simulink model "FullSystem_Electrical_Testbench"  (R2025b)
settings: Solver=ode23t  StartTime=0.0  StopTime=inf  FixedStep=Ts  MaxStep=0.0001  RelTol=1e-3
values from neighbouring files (symbols this model uses):
  servoVelocityKi = servoWn.^2.*servoJeq    [init_servos.m]
  servoVelocityKp = 2*servoZeta.*servoWn.*servoJeq    [init_servos.m]
  Ts = 0.002    [init_trajectory.m]
libraries: simulink x2
settings Model: SimulationMode=accelerator  Creator=Compu  LastModifiedBy=Compu
settings SolverCC: ZeroCrossAlgorithm=Adaptive
settings DebuggingCC: UnconnectedInputMsg=warning  UnconnectedOutputMsg=warning  UnconnectedLineMsg=warning
settings ExplorerConfigSet: SimMechanicsOpenEditorOnUpdate=off

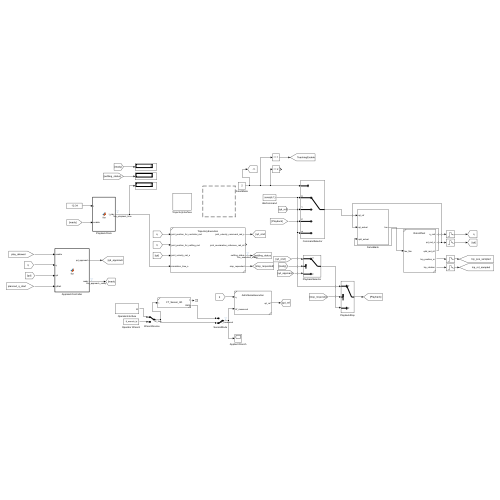
[thumbnail: Simulink's stored preview of the top-level diagram]
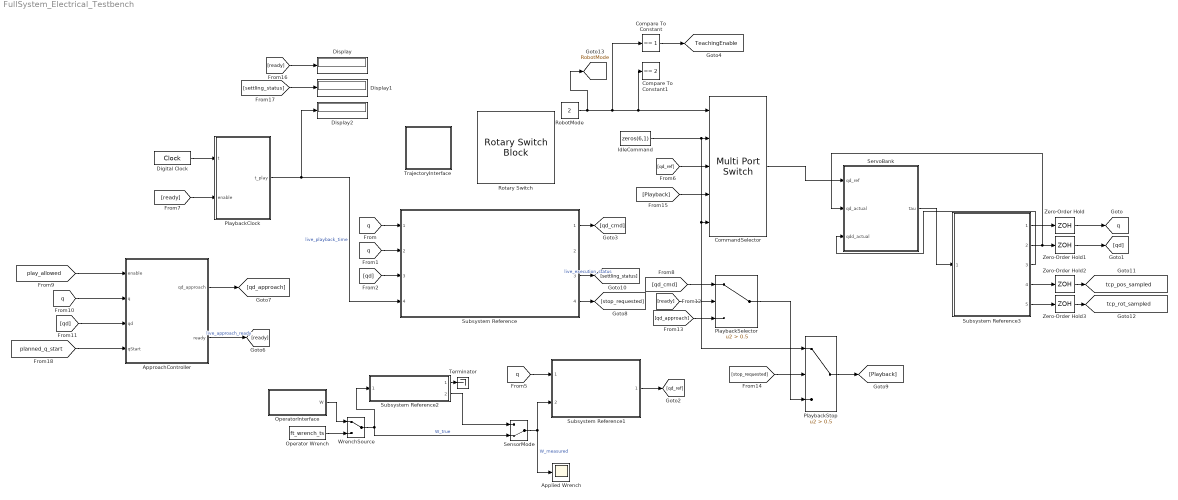
== system FullSystem_Electrical_Testbench ==
  Applied Wrench : Scope
      settings: DataLoggingVariableName=ScopeData3
  ApproachController : MATLAB Function  TreatAsAtomicUnit=on
  CommandSelector : MultiPortSwitch  DataPortOrder=Zero-based contiguous  DataPortForDefault=Additional data port  zeroidx=on  SaturateOnIntegerOverflow=off  InputSameDT=off
  Compare To Constant : simulink/Logic and Bit Operations/Compare To Constant  relop===  const=1  OutDataTypeStr=boolean
  Compare To Constant1 : simulink/Logic and Bit Operations/Compare To Constant  relop===  const=2  OutDataTypeStr=boolean
  Digital Clock : DigitalClock  SampleTime=Ts
  Display : Display
  Display1 : Display
  Display2 : Display
  IdleCommand : Constant  Value=zeros(6,1)  SampleTime=Ts
  Operator Wrench : FromWorkspace  VariableName=ft_wrench_ts  SampleTime=Ts  Interpolate=off  OutputAfterFinalValue=Holding final value
  OperatorInterface : Subsystem
  PlaybackClock : MATLAB Function  TreatAsAtomicUnit=on
  PlaybackSelector : Switch  Criteria=u2 > Threshold  Threshold=0.5  SaturateOnIntegerOverflow=off  InputSameDT=off
  PlaybackStop : Switch  Criteria=u2 > Threshold  Threshold=0.5  SaturateOnIntegerOverflow=off  InputSameDT=off
  RobotMode : Constant  Value=2  SampleTime=Ts
  Rotary Switch : RotarySwitchBlock
  SensorMode : ManualSwitch  CurrentSetting=0
  ServoBank : Subsystem
  Subsystem Reference : Subsystem  ReferencedSubsystem=TrajectoryExecution
  Subsystem Reference1 : Subsystem  ReferencedSubsystem=AdmittanceExecution
  Subsystem Reference2 : Subsystem  ReferencedSubsystem=FT_Sensor_6D
  Subsystem Reference3 : Subsystem  ReferencedSubsystem=RobotPlant
  Terminator : Terminator
  TrajectoryInterface : Subsystem
  WrenchSource : ManualSwitch
  Zero-Order Hold{,1..3} (4 alike) : ZeroOrderHold  SampleTime=Ts
  tag scope: RobotMode=global, TeachingEnable=global, q=global, tcp_pos_sampled=global, tcp_rot_sampled=global
  wires:
  Subsystem Reference2/2 -> SensorMode/1
  SensorMode/1 -> Subsystem Reference1/2, Applied Wrench/1  "W_measured"
  OperatorInterface/1(W) -> WrenchSource/1
  WrenchSource/1 -> SensorMode/2, Subsystem Reference2/1  "W_true"
  Subsystem Reference2/1 -> Terminator/1
  Operator Wrench/1 -> WrenchSource/2
  ServoBank/1(tau) -> Subsystem Reference3/1
  Subsystem Reference3/1 -> Zero-Order Hold/1
  Subsystem Reference3/2 -> ServoBank/2(qd_actual), Zero-Order Hold1/1
  Zero-Order Hold/1 -> [q]
  Zero-Order Hold1/1 -> [qd]
  [q] -> Subsystem Reference/1
  [q] -> Subsystem Reference/2
  [qd] -> Subsystem Reference/3
  [q] -> Subsystem Reference1/1
  RobotMode/1 -> [RobotMode], Compare To Constant/1, Compare To Constant1/1, CommandSelector/1
  Subsystem Reference1/1 -> [qd_ref]
  Subsystem Reference/1 -> [qd_cmd]
  [qd_ref] -> CommandSelector/3
  CommandSelector/1 -> ServoBank/1(qd_ref)
  Compare To Constant/1 -> [TeachingEnable]
  PlaybackClock/1(t_play) -> Display2/1, Subsystem Reference/4  "live_playback_time"
  Digital Clock/1 -> PlaybackClock/1(t)
  [q] -> ApproachController/2(q)
  [qd] -> ApproachController/3(qd)
  [play_allowed] -> ApproachController/1(enable)
  [planned_q_start] -> ApproachController/4(qStart)
  [qd_cmd] -> PlaybackSelector/1
  ApproachController/2(ready) -> [ready]  "live_approach_ready"
  ApproachController/1(qd_approach) -> [qd_approach]
  [ready] -> PlaybackClock/2(enable)
  [ready] -> PlaybackSelector/2
  [qd_approach] -> PlaybackSelector/3
  IdleCommand/1 -> CommandSelector/2, CommandSelector/5, PlaybackStop/1
  Subsystem Reference/4 -> [stop_requested]
  [stop_requested] -> PlaybackStop/2
  PlaybackSelector/1 -> PlaybackStop/3
  PlaybackStop/1 -> [Playback]
  [Playback] -> CommandSelector/4
  Subsystem Reference/3 -> [settling_status]  "live_execution_status"
  [ready] -> Display/1
  [settling_status] -> Display1/1
  Subsystem Reference3/4 -> Zero-Order Hold2/1
  Subsystem Reference3/5 -> Zero-Order Hold3/1
  Zero-Order Hold2/1 -> [tcp_pos_sampled]
  Zero-Order Hold3/1 -> [tcp_rot_sampled]
  Subsystem Reference3/3 -> ServoBank/3(qdd_actual)

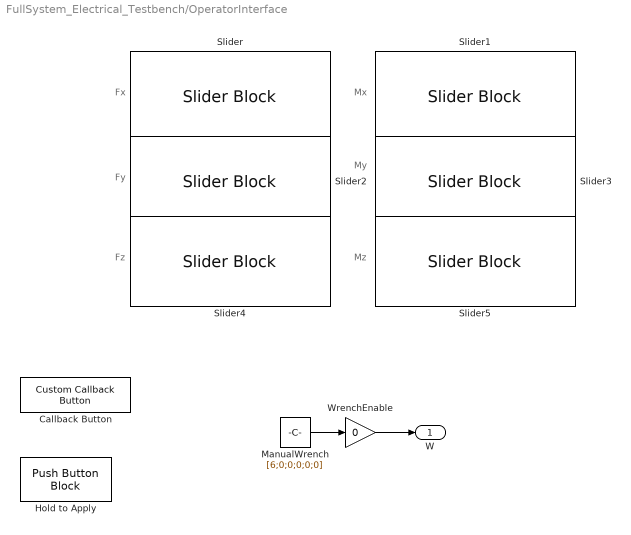
== system FullSystem_Electrical_Testbench/OperatorInterface ==
  note: Fx
  note: Fy
  note: Fz
  note: Mx
  note: My
  note: Mz
  Callback Button : CustomCallbackButton  Configuration="{\"components\":[{\"name\":\"BackgroundImageComponent\",\"settings\":{\"image\":{\"size\":[0,0],\"src\":\"default\",\"srcOrientation\":\"Right\"},\"position\":[0,0,1,1]}},{\"name\":\"ButtonStateComponent\",\"settings\":{\"buttonType\":\"momentary\",\"clickFcn\":\"set_param([get_param(gcb,'Parent') '\\/ManualWrench'], 'Value', '[0;0;0;0;0;0]');\",\"onValue\":1,\"position\":[0,0,1,1],\"pressDelay\":\"500\",\"pressFcn\":\"\",\"repeatInterval\":\"0\",\"states\":[{\"horizontalAlignment\":\"center\",\"image\":{\"position\":[0,0,1,1],\"size\":[1,1],\"src\":\"default\",\"srcOrientation\":\"Right\"},\"label\":{\"color\":[0.01176470588,0.01176470588,0.01176470588,1],\"icon\":{\"size\":[0,0],\"src\":\"default\",\"srcOrientation\":\"Right\"},\"iconOffset\":0,\"iconPlacement\":\"left\",\"opacity\":1,\"show\":true,\"text\":{\"content\":\"Reset All\",\"font\":\"Helvetica\"}},\"labelOffset\":[0,0],\"verticalAlignment\":\"middle\"},{\"horizontalAlignment\":\"center\",\"image\":{\"position\":[0,0,1,1],\"size\":[1,1],\"src\":\"default\",\"srcOrientation\":\"Right\"},\"label\":{\"color\":[0.01176470588,0.01176470588,0.01176470588,1],\"icon\":{\"size\":[0,0],\"src\":\"default\",\"srcOrientation\":\"Right\"},\"iconOffset\":0,\"iconPlacement\":\"left\",\"opacity\":1,\"show\":true,\"text\":{\"content\":\"Reset All\",\"font\":\"Helvetica\"}},\"labelOffset\":[0,0],\"verticalAlignment\":\"middle\"},{\"horizontalAlignment\":\"center\",\"image\":{\"position\":[0,0,1,1],\"size\":[1,1],\"src\":\"default\",\"srcOrientation\":\"Right\"},\"label\":{\"color\":[0.01176470588,0.01176470588,0.01176470588,1],\"icon\":{\"size\":[0,0],\"src\":\"default\",\"srcOrientation\":\"Right\"},\"iconOffset\":0,\"iconPlacement\":\"left\",\"opacity\":1,\"show\":true,\"text\":{\"content\":\"Reset All\",\"font\":\"Helvetica\"}},\"labelOffset\":[0,0],\"verticalAlignment\":\"middle\"},{\"horizontalAlignment\":\"center\",\"image\":{\"position\":[0,0,1,1],\"size\":[1,1],\"src\":\"default\",\"srcOrientation\":\"Right\"},\"label\":{\"color\":[0.01176470588,0.01176470588,0.01176470588,1],\"icon\":{\"size\":[0,0],\"src\":\"default\",\"srcOrientation\":\"Right\"},\"iconOffset\":0,\"iconPlacement\":\"left\",\"opacity\":1,\"show\":true,\"text\":{\"content\":\"Reset All\",\"font\":\"Helvetica\"}},\"labelOffset\":[0,0],\"verticalAlignment\":\"middle\"}]}},{\"name\":\"ForegroundImageComponent\",\"settings\":{\"image\":{\"size\":[0,0],\"src\":\"default\",\"srcOrientation\":\"Right\"},\"isForeground\":1,\"position\":[0,0,1,1]}}],\"derived\":{\"blockParameters\":{\"AutoActivate\":true,\"ButtonText\":\"Reset All\",\"ButtonType\":\"Momentary\",\"ClickFcn\":\"set_param([get_param(gcb,'Parent') '\\/ManualWrench'], 'Value', '[0;0;0;0;0;0]');\",\"OnValue\":1,\"PressDelay\":\"500\",\"PressFcn\":\"\",\"RepeatInterval\":\"0\",\"fixedAspectRatio\":\"off\"}},\"settings\":{\"BindingType\":\"standalone\",\"autoActivate\":true,\"backgroundColor\":[244,244,244,1],\"backgroundOffset\":0.2,\"backgroundOpacity\":1,\"fixedAspectRatio\":\"off\",\"foregroundColor\":[0.01176470588,0.01176470588,0.01176470588,1],\"migratedFromLegacy\":true,\"useBackgroundColor\":true,\"variant\":\"callback\",\"version\":\"R2025a\"},\"type\":\"Button\"}"  CustomBackgroundColor="{\"color\":[0.9568627451,0.9568627451,0.9568627451],\"show\":true}"
  Hold to Apply : PushButtonBlock  ButtonText=Hold to Apply  IconOnColor=[0.0, 0.39215686274509803, 0.0]  IconOffColor=[0.0, 1.0, 0.0]  OffValue=0.000000
  ManualWrench : Constant  Value=[6;0;0;0;0;0]  SampleTime=Ts
  Slider : SliderBlock  ScaleMin=-10  ScaleMax=10  TickInterval=5
  Slider1 : SliderBlock  ScaleMin=-1  ScaleMax=1  TickInterval=0.5
  Slider2 : SliderBlock  ScaleMin=-10  ScaleMax=10  TickInterval=5
  Slider3 : SliderBlock  ScaleMin=-1  ScaleMax=1  TickInterval=0.5
  Slider4 : SliderBlock  ScaleMin=-10  ScaleMax=10  TickInterval=5
  Slider5 : SliderBlock  ScaleMin=-1  ScaleMax=1  TickInterval=0.5
  WrenchEnable : Gain  Gain=0
  W : Outport
  wires:
  ManualWrench/1 -> WrenchEnable/1
  WrenchEnable/1 -> W/1

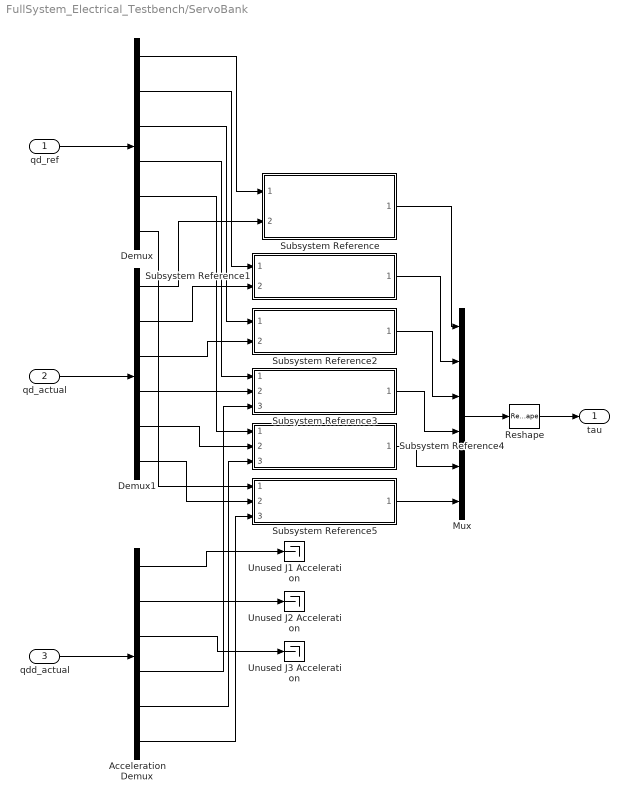
== system FullSystem_Electrical_Testbench/ServoBank ==
  qd_ref : Inport
  qd_actual : Inport  Port=2
  qdd_actual : Inport  Port=3
  Acceleration Demux : Demux  Outputs=6
  Demux : Demux  Outputs=6
  Demux1 : Demux  Outputs=6
  Mux : Mux  Inputs=6
  Reshape : Reshape  OutputDimensionality=Column vector (2-D)
  Subsystem Reference : Subsystem  ReferencedSubsystem=M8010_Actuator  VelKp=servoVelocityKp(1)  VelKi=servoVelocityKi(1)
  Subsystem Reference1 : Subsystem  ReferencedSubsystem=M8025_Actuator  VelKp=servoVelocityKp(2)  VelKi=servoVelocityKi(2)
  Subsystem Reference2 : Subsystem  ReferencedSubsystem=M8010_Actuator  VelKp=servoVelocityKp(3)  VelKi=servoVelocityKi(3)
  Subsystem Reference3 : Subsystem  ReferencedSubsystem=M6030G9_Actuator  VelKp=servoVelocityKp(4)  VelKi=servoVelocityKi(4)
  Subsystem Reference4 : Subsystem  ReferencedSubsystem=M6030G9_Actuator  VelKp=servoVelocityKp(5)  VelKi=servoVelocityKi(5)
  Subsystem Reference5 : Subsystem  ReferencedSubsystem=M6030G9_Actuator  VelKp=servoVelocityKp(6)  VelKi=servoVelocityKi(6)
  Unused J1 Acceleration : Terminator
  Unused J2 Acceleration : Terminator
  Unused J3 Acceleration : Terminator
  tau : Outport
  wires:
  Demux/3 -> Subsystem Reference2/1
  Acceleration Demux/3 -> Unused J3 Acceleration/1
  Demux/2 -> Subsystem Reference1/1
  Demux/1 -> Subsystem Reference/1
  qd_actual/1 -> Demux1/1
  qd_ref/1 -> Demux/1
  qdd_actual/1 -> Acceleration Demux/1
  Demux/5 -> Subsystem Reference4/1
  Demux/4 -> Subsystem Reference3/1
  Acceleration Demux/2 -> Unused J2 Acceleration/1
  Demux/6 -> Subsystem Reference5/1
  Demux1/1 -> Subsystem Reference/2
  Subsystem Reference4/1 -> Mux/5
  Demux1/2 -> Subsystem Reference1/2
  Demux1/3 -> Subsystem Reference2/2
  Demux1/4 -> Subsystem Reference3/2
  Demux1/5 -> Subsystem Reference4/2
  Demux1/6 -> Subsystem Reference5/2
  Subsystem Reference/1 -> Mux/1
  Acceleration Demux/1 -> Unused J1 Acceleration/1
  Acceleration Demux/4 -> Subsystem Reference3/3
  Acceleration Demux/5 -> Subsystem Reference4/3
  Acceleration Demux/6 -> Subsystem Reference5/3
  Subsystem Reference1/1 -> Mux/2
  Subsystem Reference2/1 -> Mux/3
  Subsystem Reference3/1 -> Mux/4
  Subsystem Reference5/1 -> Mux/6
  Mux/1 -> Reshape/1
  Reshape/1 -> tau/1

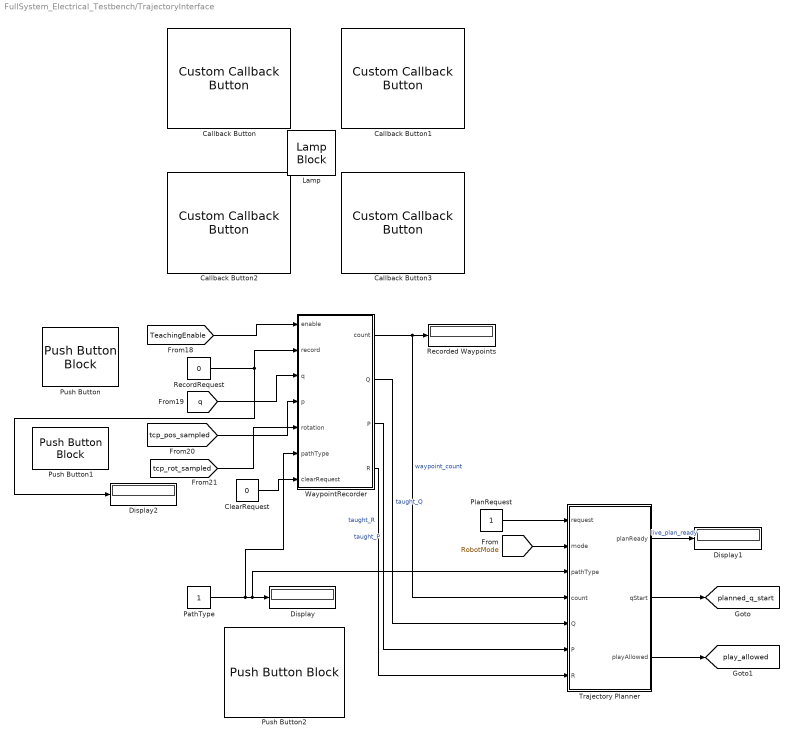
== system FullSystem_Electrical_Testbench/TrajectoryInterface ==
  Callback Button : CustomCallbackButton  Configuration="{\"components\":[{\"name\":\"BackgroundImageComponent\",\"settings\":{\"image\":{\"size\":[0,0],\"src\":\"default\",\"srcOrientation\":\"Right\"},\"position\":[0,0,1,1]}},{\"name\":\"ButtonStateComponent\",\"settings\":{\"buttonType\":\"momentary\",\"clickFcn\":\"set_param('FullSystem_Electrical_Testbench\\/TrajectoryInterface\\/PathType','Value','1');\",\"onValue\":1,\"position\":[0,0,1,1],\"pressDelay\":\"500\",\"pressFcn\":\"\",\"repeatInterval\":\"0\",\"states\":[{\"horizontalAlignment\":\"center\",\"image\":{\"position\":[0,0,1,1],\"size\":[1,1],\"src\":\"default\",\"srcOrientation\":\"Right\"},\"label\":{\"color\":[0.7490196078431373,0.33725490196078434,0.33725490196078434],\"icon\":{\"size\":[0,0],\"src\":\"default\",\"srcOrientation\":\"Right\"},\"iconOffset\":0,\"iconPlacement\":\"left\",\"opacity\":1,\"show\":true,\"text\":{\"content\":\"Straight Line\",\"font\":\"Helvetica\"}},\"labelOffset\":[0,0],\"verticalAlignment\":\"middle\"},{\"horizontalAlignment\":\"center\",\"image\":{\"position\":[0,0,1,1],\"size\":[1,1],\"src\":\"default\",\"srcOrientation\":\"Right\"},\"label\":{\"color\":[0.01176470588,0.01176470588,0.01176470588,1],\"icon\":{\"size\":[0,0],\"src\":\"default\",\"srcOrientation\":\"Right\"},\"iconOffset\":0,\"iconPlacement\":\"left\",\"opacity\":1,\"show\":true,\"text\":{\"content\":\"Straight Line\",\"font\":\"Helvetica\"}},\"labelOffset\":[0,0],\"verticalAlignment\":\"middle\"},{\"horizontalAlignment\":\"center\",\"image\":{\"position\":[0,0,1,1],\"size\":[1,1],\"src\":\"default\",\"srcOrientation\":\"Right\"},\"label\":{\"color\":[0.01176470588,0.01176470588,0.01176470588,1],\"icon\":{\"size\":[0,0],\"src\":\"default\",\"srcOrientation\":\"Right\"},\"iconOffset\":0,\"iconPlacement\":\"left\",\"opacity\":1,\"show\":true,\"text\":{\"content\":\"Straight Line\",\"font\":\"Helvetica\"}},\"labelOffset\":[0,0],\"verticalAlignment\":\"middle\"},{\"horizontalAlignment\":\"center\",\"image\":{\"position\":[0,0,1,1],\"size\":[1,1],\"src\":\"default\",\"srcOrientation\":\"Right\"},\"label\":{\"color\":[0.01176470588,0.01176470588,0.01176470588,1],\"icon\":{\"size\":[0,0],\"src\":\"default\",\"srcOrientation\":\"Right\"},\"iconOffset\":0,\"iconPlacement\":\"left\",\"opacity\":1,\"show\":true,\"text\":{\"content\":\"Straight Line\",\"font\":\"Helvetica\"}},\"labelOffset\":[0,0],\"verticalAlignment\":\"middle\"}]}},{\"name\":\"ForegroundImageComponent\",\"settings\":{\"image\":{\"size\":[0,0],\"src\":\"default\",\"srcOrientation\":\"Right\"},\"isForeground\":1,\"position\":[0,0,1,1]}}],\"derived\":{\"blockParameters\":{\"AutoActivate\":true,\"ButtonText\":\"Straight Line\",\"ButtonType\":\"Momentary\",\"ClickFcn\":\"set_param('FullSystem_Electrical_Testbench\\/TrajectoryInterface\\/PathType','Value','1');\",\"OnValue\":1,\"PressDelay\":\"500\",\"PressFcn\":\"\",\"RepeatInterval\":\"0\",\"fixedAspectRatio\":\"off\"}},\"settings\":{\"BindingType\":\"standalone\",\"autoActivate\":true,\"backgroundColor\":[244,244,244,1],\"backgroundOffset\":0.2,\"backgroundOpacity\":1,\"fixedAspectRatio\":\"off\",\"foregroundColor\":[0.01176470588,0.01176470588,0.01176470588,1],\"migratedFromLegacy\":true,\"useBackgroundColor\":true,\"variant\":\"callback\",\"version\":\"R2025a\"},\"type\":\"Button\"}"  CustomBackgroundColor="{\"color\":[0.9568627451,0.9568627451,0.9568627451],\"show\":true}"
  Callback Button1 : CustomCallbackButton  Configuration="{\"components\":[{\"name\":\"BackgroundImageComponent\",\"settings\":{\"image\":{\"size\":[0,0],\"src\":\"default\",\"srcOrientation\":\"Right\"},\"position\":[0,0,1,1]}},{\"name\":\"ButtonStateComponent\",\"settings\":{\"buttonType\":\"momentary\",\"clickFcn\":\"set_param('FullSystem_Electrical_Testbench\\/TrajectoryInterface\\/PathType','Value','2');\\n\",\"onValue\":1,\"position\":[0,0,1,1],\"pressDelay\":\"500\",\"pressFcn\":\"\",\"repeatInterval\":\"0\",\"states\":[{\"horizontalAlignment\":\"center\",\"image\":{\"position\":[0,0,1,1],\"size\":[1,1],\"src\":\"default\",\"srcOrientation\":\"Right\"},\"label\":{\"color\":[0.7490196078431373,0.33725490196078434,0.33725490196078434],\"icon\":{\"size\":[0,0],\"src\":\"default\",\"srcOrientation\":\"Right\"},\"iconOffset\":0,\"iconPlacement\":\"left\",\"opacity\":1,\"show\":true,\"text\":{\"content\":\"Circular Arc\",\"font\":\"Helvetica\"}},\"labelOffset\":[0,0],\"verticalAlignment\":\"middle\"},{\"horizontalAlignment\":\"center\",\"image\":{\"position\":[0,0,1,1],\"size\":[1,1],\"src\":\"default\",\"srcOrientation\":\"Right\"},\"label\":{\"color\":[0.01176470588,0.01176470588,0.01176470588,1],\"icon\":{\"size\":[0,0],\"src\":\"default\",\"srcOrientation\":\"Right\"},\"iconOffset\":0,\"iconPlacement\":\"left\",\"opacity\":1,\"show\":true,\"text\":{\"content\":\"Circular Arc\",\"font\":\"Helvetica\"}},\"labelOffset\":[0,0],\"verticalAlignment\":\"middle\"},{\"horizontalAlignment\":\"center\",\"image\":{\"position\":[0,0,1,1],\"size\":[1,1],\"src\":\"default\",\"srcOrientation\":\"Right\"},\"label\":{\"color\":[0.01176470588,0.01176470588,0.01176470588,1],\"icon\":{\"size\":[0,0],\"src\":\"default\",\"srcOrientation\":\"Right\"},\"iconOffset\":0,\"iconPlacement\":\"left\",\"opacity\":1,\"show\":true,\"text\":{\"content\":\"Circular Arc\",\"font\":\"Helvetica\"}},\"labelOffset\":[0,0],\"verticalAlignment\":\"middle\"},{\"horizontalAlignment\":\"center\",\"image\":{\"position\":[0,0,1,1],\"size\":[1,1],\"src\":\"default\",\"srcOrientation\":\"Right\"},\"label\":{\"color\":[0.01176470588,0.01176470588,0.01176470588,1],\"icon\":{\"size\":[0,0],\"src\":\"default\",\"srcOrientation\":\"Right\"},\"iconOffset\":0,\"iconPlacement\":\"left\",\"opacity\":1,\"show\":true,\"text\":{\"content\":\"Circular Arc\",\"font\":\"Helvetica\"}},\"labelOffset\":[0,0],\"verticalAlignment\":\"middle\"}]}},{\"name\":\"ForegroundImageComponent\",\"settings\":{\"image\":{\"size\":[0,0],\"src\":\"default\",\"srcOrientation\":\"Right\"},\"isForeground\":1,\"position\":[0,0,1,1]}}],\"derived\":{\"blockParameters\":{\"AutoActivate\":true,\"ButtonText\":\"Circular Arc\",\"ButtonType\":\"Momentary\",\"ClickFcn\":\"set_param('FullSystem_Electrical_Testbench\\/TrajectoryInterface\\/PathType','Value','2');\\n\",\"OnValue\":1,\"PressDelay\":\"500\",\"PressFcn\":\"\",\"RepeatInterval\":\"0\",\"fixedAspectRatio\":\"off\"}},\"settings\":{\"BindingType\":\"standalone\",\"autoActivate\":true,\"backgroundColor\":[244,244,244,1],\"backgroundOffset\":0.2,\"backgroundOpacity\":1,\"fixedAspectRatio\":\"off\",\"foregroundColor\":[0.01176470588,0.01176470588,0.01176470588,1],\"migratedFromLegacy\":true,\"useBackgroundColor\":true,\"variant\":\"callback\",\"version\":\"R2025a\"},\"type\":\"Button\"}"  CustomBackgroundColor="{\"color\":[0.9568627451,0.9568627451,0.9568627451],\"show\":true}"
  Callback Button2 : CustomCallbackButton  Configuration="{\"components\":[{\"name\":\"BackgroundImageComponent\",\"settings\":{\"image\":{\"size\":[0,0],\"src\":\"default\",\"srcOrientation\":\"Right\"},\"position\":[0,0,1,1]}},{\"name\":\"ButtonStateComponent\",\"settings\":{\"buttonType\":\"momentary\",\"clickFcn\":\"set_param('FullSystem_Electrical_Testbench\\/TrajectoryInterface\\/PathType','Value','3');\\n\",\"onValue\":1,\"position\":[0,0,1,1],\"pressDelay\":\"500\",\"pressFcn\":\"\",\"repeatInterval\":\"0\",\"states\":[{\"horizontalAlignment\":\"center\",\"image\":{\"position\":[0,0,1,1],\"size\":[1,1],\"src\":\"default\",\"srcOrientation\":\"Right\"},\"label\":{\"color\":[0.7490196078431373,0.33725490196078434,0.33725490196078434],\"icon\":{\"size\":[0,0],\"src\":\"default\",\"srcOrientation\":\"Right\"},\"iconOffset\":0,\"iconPlacement\":\"left\",\"opacity\":1,\"show\":true,\"text\":{\"content\":\"Full Circle\",\"font\":\"Helvetica\"}},\"labelOffset\":[0,0],\"verticalAlignment\":\"middle\"},{\"horizontalAlignment\":\"center\",\"image\":{\"position\":[0,0,1,1],\"size\":[1,1],\"src\":\"default\",\"srcOrientation\":\"Right\"},\"label\":{\"color\":[0.01176470588,0.01176470588,0.01176470588,1],\"icon\":{\"size\":[0,0],\"src\":\"default\",\"srcOrientation\":\"Right\"},\"iconOffset\":0,\"iconPlacement\":\"left\",\"opacity\":1,\"show\":true,\"text\":{\"content\":\"Full Circle\",\"font\":\"Helvetica\"}},\"labelOffset\":[0,0],\"verticalAlignment\":\"middle\"},{\"horizontalAlignment\":\"center\",\"image\":{\"position\":[0,0,1,1],\"size\":[1,1],\"src\":\"default\",\"srcOrientation\":\"Right\"},\"label\":{\"color\":[0.01176470588,0.01176470588,0.01176470588,1],\"icon\":{\"size\":[0,0],\"src\":\"default\",\"srcOrientation\":\"Right\"},\"iconOffset\":0,\"iconPlacement\":\"left\",\"opacity\":1,\"show\":true,\"text\":{\"content\":\"Full Circle\",\"font\":\"Helvetica\"}},\"labelOffset\":[0,0],\"verticalAlignment\":\"middle\"},{\"horizontalAlignment\":\"center\",\"image\":{\"position\":[0,0,1,1],\"size\":[1,1],\"src\":\"default\",\"srcOrientation\":\"Right\"},\"label\":{\"color\":[0.01176470588,0.01176470588,0.01176470588,1],\"icon\":{\"size\":[0,0],\"src\":\"default\",\"srcOrientation\":\"Right\"},\"iconOffset\":0,\"iconPlacement\":\"left\",\"opacity\":1,\"show\":true,\"text\":{\"content\":\"Full Circle\",\"font\":\"Helvetica\"}},\"labelOffset\":[0,0],\"verticalAlignment\":\"middle\"}]}},{\"name\":\"ForegroundImageComponent\",\"settings\":{\"image\":{\"size\":[0,0],\"src\":\"default\",\"srcOrientation\":\"Right\"},\"isForeground\":1,\"position\":[0,0,1,1]}}],\"derived\":{\"blockParameters\":{\"AutoActivate\":true,\"ButtonText\":\"Full Circle\",\"ButtonType\":\"Momentary\",\"ClickFcn\":\"set_param('FullSystem_Electrical_Testbench\\/TrajectoryInterface\\/PathType','Value','3');\\n\",\"OnValue\":1,\"PressDelay\":\"500\",\"PressFcn\":\"\",\"RepeatInterval\":\"0\",\"fixedAspectRatio\":\"off\"}},\"settings\":{\"BindingType\":\"standalone\",\"autoActivate\":true,\"backgroundColor\":[244,244,244,1],\"backgroundOffset\":0.2,\"backgroundOpacity\":1,\"fixedAspectRatio\":\"off\",\"foregroundColor\":[0.01176470588,0.01176470588,0.01176470588,1],\"migratedFromLegacy\":true,\"useBackgroundColor\":true,\"variant\":\"callback\",\"version\":\"R2025a\"},\"type\":\"Button\"}"  CustomBackgroundColor="{\"color\":[0.9568627451,0.9568627451,0.9568627451],\"show\":true}"
  Callback Button3 : CustomCallbackButton  Configuration="{\"components\":[{\"name\":\"BackgroundImageComponent\",\"settings\":{\"image\":{\"size\":[0,0],\"src\":\"default\",\"srcOrientation\":\"Right\"},\"position\":[0,0,1,1]}},{\"name\":\"ButtonStateComponent\",\"settings\":{\"buttonType\":\"momentary\",\"clickFcn\":\"set_param('FullSystem_Electrical_Testbench\\/TrajectoryInterface\\/PathType','Value','4');\\n\",\"onValue\":1,\"position\":[0,0,1,1],\"pressDelay\":\"500\",\"pressFcn\":\"\",\"repeatInterval\":\"0\",\"states\":[{\"horizontalAlignment\":\"center\",\"image\":{\"position\":[0,0,1,1],\"size\":[1,1],\"src\":\"default\",\"srcOrientation\":\"Right\"},\"label\":{\"color\":[0.7490196078431373,0.33725490196078434,0.33725490196078434],\"icon\":{\"size\":[0,0],\"src\":\"default\",\"srcOrientation\":\"Right\"},\"iconOffset\":0,\"iconPlacement\":\"left\",\"opacity\":1,\"show\":true,\"text\":{\"content\":\"Multi-segment\",\"font\":\"Helvetica\"}},\"labelOffset\":[0,0],\"verticalAlignment\":\"middle\"},{\"horizontalAlignment\":\"center\",\"image\":{\"position\":[0,0,1,1],\"size\":[1,1],\"src\":\"default\",\"srcOrientation\":\"Right\"},\"label\":{\"color\":[0.01176470588,0.01176470588,0.01176470588,1],\"icon\":{\"size\":[0,0],\"src\":\"default\",\"srcOrientation\":\"Right\"},\"iconOffset\":0,\"iconPlacement\":\"left\",\"opacity\":1,\"show\":true,\"text\":{\"content\":\"Multi-segment\",\"font\":\"Helvetica\"}},\"labelOffset\":[0,0],\"verticalAlignment\":\"middle\"},{\"horizontalAlignment\":\"center\",\"image\":{\"position\":[0,0,1,1],\"size\":[1,1],\"src\":\"default\",\"srcOrientation\":\"Right\"},\"label\":{\"color\":[0.01176470588,0.01176470588,0.01176470588,1],\"icon\":{\"size\":[0,0],\"src\":\"default\",\"srcOrientation\":\"Right\"},\"iconOffset\":0,\"iconPlacement\":\"left\",\"opacity\":1,\"show\":true,\"text\":{\"content\":\"Multi-segment\",\"font\":\"Helvetica\"}},\"labelOffset\":[0,0],\"verticalAlignment\":\"middle\"},{\"horizontalAlignment\":\"center\",\"image\":{\"position\":[0,0,1,1],\"size\":[1,1],\"src\":\"default\",\"srcOrientation\":\"Right\"},\"label\":{\"color\":[0.01176470588,0.01176470588,0.01176470588,1],\"icon\":{\"size\":[0,0],\"src\":\"default\",\"srcOrientation\":\"Right\"},\"iconOffset\":0,\"iconPlacement\":\"left\",\"opacity\":1,\"show\":true,\"text\":{\"content\":\"Multi-segment\",\"font\":\"Helvetica\"}},\"labelOffset\":[0,0],\"verticalAlignment\":\"middle\"}]}},{\"name\":\"ForegroundImageComponent\",\"settings\":{\"image\":{\"size\":[0,0],\"src\":\"default\",\"srcOrientation\":\"Right\"},\"isForeground\":1,\"position\":[0,0,1,1]}}],\"derived\":{\"blockParameters\":{\"AutoActivate\":true,\"ButtonText\":\"Multi-segment\",\"ButtonType\":\"Momentary\",\"ClickFcn\":\"set_param('FullSystem_Electrical_Testbench\\/TrajectoryInterface\\/PathType','Value','4');\\n\",\"OnValue\":1,\"PressDelay\":\"500\",\"PressFcn\":\"\",\"RepeatInterval\":\"0\",\"fixedAspectRatio\":\"off\"}},\"settings\":{\"BindingType\":\"standalone\",\"autoActivate\":true,\"backgroundColor\":[244,244,244,1],\"backgroundOffset\":0.2,\"backgroundOpacity\":1,\"fixedAspectRatio\":\"off\",\"foregroundColor\":[0.01176470588,0.01176470588,0.01176470588,1],\"migratedFromLegacy\":true,\"useBackgroundColor\":true,\"variant\":\"callback\",\"version\":\"R2025a\"},\"type\":\"Button\"}"  CustomBackgroundColor="{\"color\":[0.9568627451,0.9568627451,0.9568627451],\"show\":true}"
  ClearRequest : Constant  Value=0
  Display : Display
  Display1 : Display
  Display2 : Display
  Lamp : LampBlock  LabelPosition=Hide  DefaultColor=[192.0, 192.0, 192.0]
  PathType : Constant  SampleTime=Ts
  PlanRequest : Constant  SampleTime=Ts
  Push Button : PushButtonBlock  ButtonText=Record Waypoint  IconOnColor=[0.0, 0.39215686274509803, 0.0]  IconOffColor=[0.0, 1.0, 0.0]  OffValue=0.000000
  Push Button1 : PushButtonBlock  ButtonText=Clear Waypoints  IconOnColor=[0.0, 0.39215686274509803, 0.0]  IconOffColor=[0.0, 1.0, 0.0]  OffValue=1.000000
  Push Button2 : PushButtonBlock  ButtonText=Generate Trajectory  ButtonType=Latch  IconOnColor=[0.0, 0.39215686274509803, 0.0]  IconOffColor=[0.0, 1.0, 0.0]  OffValue=0.000000
  RecordRequest : Constant  Value=0  SampleTime=Ts
  Recorded Waypoints : Display
  Trajectory Planner : MATLAB Function  TreatAsAtomicUnit=on
  WaypointRecorder : MATLAB Function  TreatAsAtomicUnit=on
  tag scope: planned_q_start=global, play_allowed=global
  wires:
  [TeachingEnable] -> WaypointRecorder/1(enable)
  WaypointRecorder/3(P) -> Trajectory Planner/6(P)  "taught_P"
  WaypointRecorder/2(Q) -> Trajectory Planner/5(Q)  "taught_Q"
  WaypointRecorder/4(R) -> Trajectory Planner/7(R)  "taught_R"
  [tcp_pos_sampled] -> WaypointRecorder/4(p)
  [tcp_rot_sampled] -> WaypointRecorder/5(rotation)
  [q] -> WaypointRecorder/3(q)
  RecordRequest/1 -> WaypointRecorder/2(record), Display2/1
  WaypointRecorder/1(count) -> Trajectory Planner/4(count), Recorded Waypoints/1  "waypoint_count"
  PathType/1 -> WaypointRecorder/6(pathType), Trajectory Planner/3(pathType), Display/1
  ClearRequest/1 -> WaypointRecorder/7(clearRequest)
  PlanRequest/1 -> Trajectory Planner/1(request)
  [RobotMode] -> Trajectory Planner/2(mode)
  Trajectory Planner/2(qStart) -> [planned_q_start]
  Trajectory Planner/3(playAllowed) -> [play_allowed]
  Trajectory Planner/1(planReady) -> Display1/1  "live_plan_ready"

== matlab function FullSystem_Electrical_Testbench/PlaybackClock ==
  data: t input; t_play output; enable input
function t_play = fcn(t, enable)

persistent tStart wasEnabled

if isempty(wasEnabled)
    tStart = t;
    wasEnabled = false;
end

if ~enable
    t_play = 0;
elseif ~wasEnabled
    tStart = t;
    t_play = 0;
else
    t_play = t - tStart;
end

wasEnabled = enable;

end

== matlab function FullSystem_Electrical_Testbench/ApproachController ==
  data: enable input; qd_approach output; q input; qd input; qStart input; ready output
function [qd_approach, ready] = fcn(enable, q, qd, qStart)

persistent reached

if isempty(reached)
    reached = false;
end

qd_approach = zeros(6,1);

if ~enable
    reached = false;
else
    if ~reached
        e = qStart(:) - q(:);

        % Bounded joint velocity command
        qd_approach = min(max(e, -0.15), 0.15);

        if max(abs(e)) <= 0.00035 && ...
           max(abs(qd(:))) <= 0.003

            reached = true;
            qd_approach = zeros(6,1);
        end
    end
end

ready = reached;

end

== matlab function FullSystem_Electrical_Testbench/TrajectoryInterface/WaypointRecorder ==
  data: enable input; count output; record input; q input; p input; rotation input; Q output; P output; R output; pathType input; clearRequest input
function [count,Q,P,R] = fcn( ...
    enable,record,q,p,rotation,pathType,clearRequest)

persistent n Qbuf Pbuf Rbuf
persistent previousRecord previousType

if isempty(n)
    n = 0;
    Qbuf = zeros(6,100);
    Pbuf = zeros(3,100);
    Rbuf = zeros(3,3,100);
    previousRecord = false;
    previousType = pathType;
end

%% Clear buffer when requested or geometry changes

if clearRequest > 0.5 || pathType ~= previousType
    n = 0;
    Qbuf(:) = 0;
    Pbuf(:) = 0;
    Rbuf(:) = 0;

else

    %% Determine waypoint capacity

    switch pathType
        case 1
            maxPoints = 2;
        case {2,3}
            maxPoints = 3;
        case 4
            maxPoints = 100;
        otherwise
            maxPoints = 0;
    end

    %% Record waypoint

    pressed = record > 0.5;

    if enable && pressed && ~previousRecord ...
            && n < maxPoints

        n = n + 1;
        Qbuf(:,n) = q(:);
        Pbuf(:,n) = p(:);
        Rbuf(:,:,n) = reshape(rotation,3,3);

    end
end

previousRecord = record > 0.5;
previousType = pathType;

count = n;
Q = Qbuf;
P = Pbuf;
R = Rbuf;

end

== matlab function FullSystem_Electrical_Testbench/TrajectoryInterface/Trajectory Planner ==
  data: request input; planReady output; mode input; pathType input; count input; Q input; P input; R input; qStart output; playAllowed output
function [planReady,qStart,playAllowed] = ...
    fcn(request,mode,pathType,count,Q,P,R)

coder.extrinsic('plan_taught_trajectory');

persistent valid startQ previousRequest
persistent previousCount previousType

if isempty(valid)
    valid = false;
    startQ = zeros(6,1);
    previousRequest = false;
    previousCount = -1;
    previousType = -1;
end

% Invalidate old plan when waypoints change
if count ~= previousCount || pathType ~= previousType
    valid = false;
end

pressed = request > 0.5;

% Only generate a trajectory in IDLE
if pressed && ~previousRequest && mode == 0
    [valid,startQ] = ...
        plan_taught_trajectory(pathType,count,Q,P,R);
end

previousRequest = pressed;
previousCount = count;
previousType = pathType;

planReady = valid;
qStart = startQ;
playAllowed = mode == 2 && valid;

end
